simulink model "rsw_demo_robot"  (Simulink 8.0)
Description:
  | generated by rsw-audit

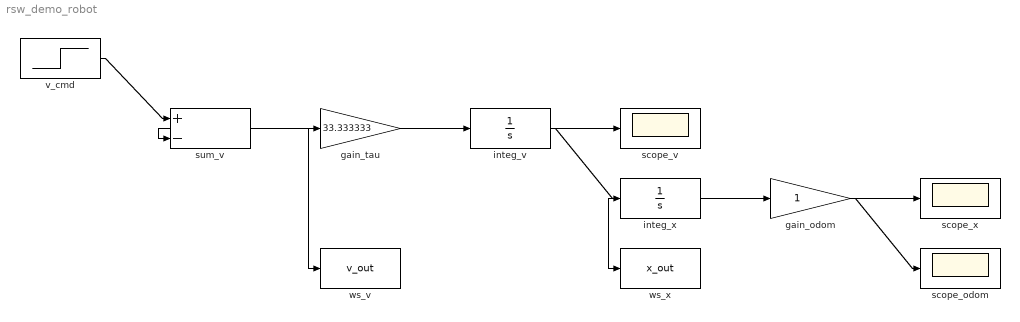
== system rsw_demo_robot ==
  v_cmd : Step  Time=0  Before=0  After=0.3
  sum_v : Sum  Inputs=+-
  gain_tau : Gain  Gain=33.333333
  integ_v : Integrator  InitialCondition=0
  integ_x : Integrator  InitialCondition=0
  gain_odom : Gain  Gain=1
  scope_v : Scope
  scope_x : Scope
  scope_odom : Scope
  ws_v : ToWorkspace  VariableName=v_out  SaveFormat=Array
  ws_x : ToWorkspace  VariableName=x_out  SaveFormat=Array
  wires:
  v_cmd/1 -> sum_v/1
  integ_v/1 -> sum_v/2
  sum_v/1 -> gain_tau/1
  gain_tau/1 -> integ_v/1
  integ_v/1 -> ws_v/1
  integ_x/1 -> ws_x/1
  integ_v/1 -> integ_x/1
  integ_v/1 -> scope_v/1
  integ_x/1 -> scope_x/1
  integ_x/1 -> gain_odom/1
  gain_odom/1 -> scope_odom/1
